simulink model "mdl_VD_st2dof_R2025b_SLX"  (R2025b)
settings: Solver=ode3  StartTime=startTime  StopTime=endTime  FixedStep=deltaT  MaxStep=deltaT  RelTol=1e-3  EnableMultiTasking=on
values from neighbouring files (symbols this model uses):
  initialStates = [0 0 0 0 0]    [script_test_fcn_VD_st2dofSimulink.m]
  parameters = struct    [fcn_VD_st2dofSimulink.m]
  U = 20    [script_test_fcn_VD_st2dofSimulink.m]
settings Model: Creator=snb10  LastModifiedBy=snb10
settings SolverCC: AlgebraicLoopSolver=TrustRegion
settings DataIOCC: LimitDataPoints=on  SaveFormat=Array  SignalLoggingSaveFormat=ModelDataLogs  ReturnWorkspaceOutputs=off  SignalLoggingName=sigsOut
settings OptimizationCC: InitFltsAndDblsToZero=on  LifeSpan=inf
settings DebuggingCC: SaveWithParameterizedLinksMsg=none  UnderspecifiedInitializationDetection=Classic  MergeDetectMultiDrivingBlocksExec=none  SignalResolutionControl=TryResolveAllWithWarning  MultiTaskDSMMsg=warning  MultiTaskCondExecSysMsg=none  FcnCallInpInsideContextMsg=warning  UnconnectedInputMsg=warning  UnconnectedOutputMsg=warning  UnconnectedLineMsg=warning  StateNameClashWarn=warning  SFUnexpectedBacktrackingDiag=warning  SFNoUnconditionalDefaultTransitionDiag=warning  SFExecutionAtInitializationDiag=none  ArithmeticOperatorsInVariantConditions=warning
settings HardwareCC: ProdBitPerPointer=32.0  ProdBitPerSizeT=32.0  ProdBitPerPtrDiffT=32.0  ProdLargestAtomicFloat=None  ProdIntDivRoundTo=Undefined  ProdEndianess=Unspecified  ProdWordSize=32.0  ProdHWDeviceType=32-bit Generic  TargetUnknown=on
settings ModelReferenceCC: EnableRefExpFcnMdlSchedulingChecks=on  PropagateSignalLabelsOutOfModel=off
settings SFSimCC: SimUseLocalCustomCode=off  CustomCodeUndefinedFunction=UseInterfaceOnly
settings RTWCC: RTWUseLocalCustomCode=off  GPUComputeCapability=3.5  DLArmComputeVersion=19.05
settings CodeAppCC: StateflowObjectComments=on
settings GRTTargetCC: TargetFcnLib=ansi_tfl_tmw.mat  TargetLangStandard=C89/C90 (ANSI)  CombineOutputUpdateFcns=off  GRTInterface=on
settings ConfigComp: CovMetricSettings=dw  CovSaveCumulativeToWorkspaceVar=on  CovSaveSingleToWorkspaceVar=on  CovExternalEMLEnable=off

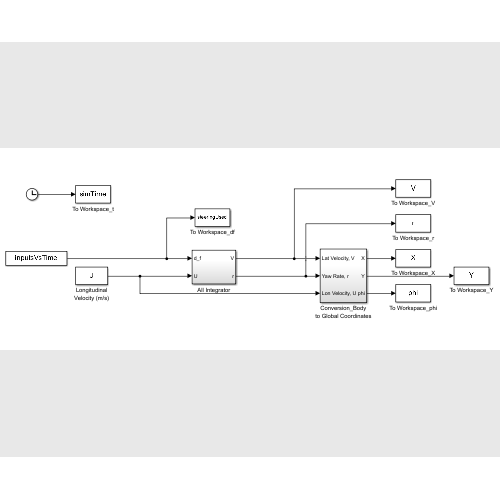
[thumbnail: Simulink's stored preview of the top-level diagram]
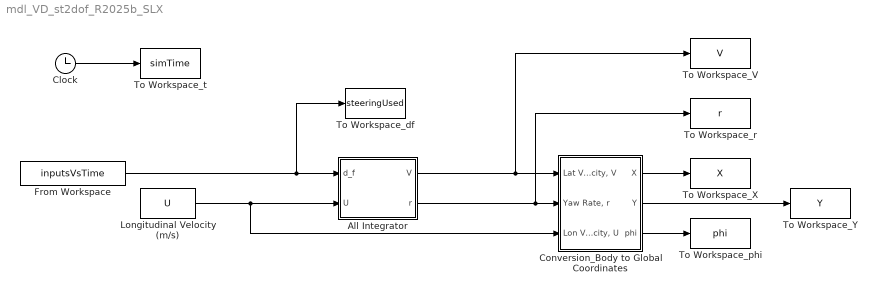
== system mdl_VD_st2dof_R2025b_SLX ==
  All Integrator : Subsystem
  Clock : Clock
  Conversion_Body to Global Coordinates : Subsystem
  From Workspace : FromWorkspace  VariableName=inputsVsTime  OutDataTypeStr=double  SampleTime=.01  OutputAfterFinalValue=Holding final value
  Longitudinal Velocity (m/s) : Constant  Value=U
  To Workspace_V : ToWorkspace  VariableName=V  SampleTime=-1
  To Workspace_X : ToWorkspace  VariableName=X  SampleTime=-1
  To Workspace_Y : ToWorkspace  VariableName=Y  SampleTime=-1
  To Workspace_df : ToWorkspace  VariableName=steeringUsed  SampleTime=-1
  To Workspace_phi : ToWorkspace  VariableName=phi  SampleTime=-1
  To Workspace_r : ToWorkspace  VariableName=r  SampleTime=-1
  To Workspace_t : ToWorkspace  VariableName=simTime  SampleTime=-1
  wires:
  Clock/1 -> To Workspace_t/1
  All Integrator/1(V) -> Conversion_Body to Global Coordinates/1("Lat Velocity, V"), To Workspace_V/1
  Conversion_Body to Global Coordinates/1(X) -> To Workspace_X/1
  Conversion_Body to Global Coordinates/2(Y) -> To Workspace_Y/1
  All Integrator/2(r) -> Conversion_Body to Global Coordinates/2("Yaw Rate, r"), To Workspace_r/1
  Conversion_Body to Global Coordinates/3(phi) -> To Workspace_phi/1
  Longitudinal Velocity (m/s)/1 -> Conversion_Body to Global Coordinates/3("Lon Velocity, U"), All Integrator/2(U)
  From Workspace/1 -> To Workspace_df/1, All Integrator/1(d_f)

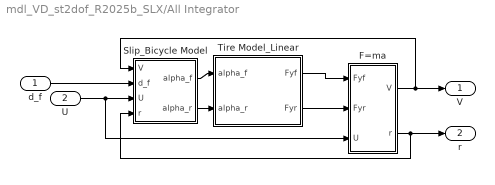
== system mdl_VD_st2dof_R2025b_SLX/All Integrator ==
  d_f : Inport
  U : Inport  Port=2
  F=ma : Subsystem
  Slip_Bicycle Model : Subsystem
  Tire Model_Linear : Subsystem
  V : Outport
  r : Outport  Port=2
  wires:
  Slip_Bicycle Model/1(alpha_f) -> Tire Model_Linear/1(alpha_f)
  Slip_Bicycle Model/2(alpha_r) -> Tire Model_Linear/2(alpha_r)
  Tire Model_Linear/1(Fyf) -> F=ma/1(Fyf)
  Tire Model_Linear/2(Fyr) -> F=ma/2(Fyr)
  U/1 -> Slip_Bicycle Model/3(U), F=ma/3(" U")
  d_f/1 -> Slip_Bicycle Model/2(d_f)
  F=ma/1(V) -> V/1, Slip_Bicycle Model/1(V)
  F=ma/2(r) -> r/1, Slip_Bicycle Model/4(r)

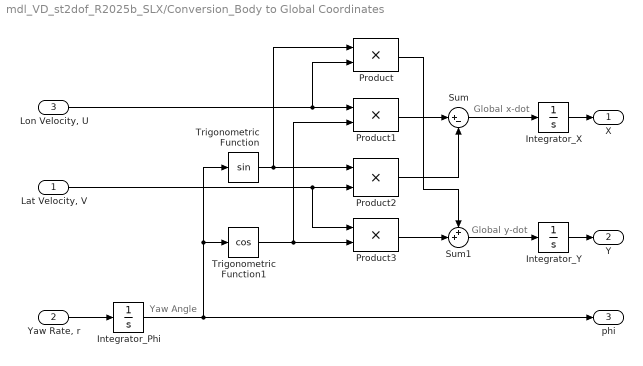
== system mdl_VD_st2dof_R2025b_SLX/Conversion_Body to Global Coordinates ==
  note: Global y-dot
  note: Global x-dot
  note: Yaw Angle
  "Lat Velocity, V" : Inport
  "Yaw Rate, r" : Inport  Port=2
  "Lon Velocity, U" : Inport  Port=3
  Integrator_Phi : Integrator  InitialCondition=initialStates(5)
  Integrator_X : Integrator  InitialCondition=initialStates(3)
  Integrator_Y : Integrator  InitialCondition=initialStates(4)
  Product{,1..3} (4 alike) : Product  SaturateOnIntegerOverflow=on  OutDataTypeStr=Inherit: Same as first input
  Sum : Sum  Inputs=|+-  SaturateOnIntegerOverflow=on
  Sum1 : Sum  Inputs=++|  SaturateOnIntegerOverflow=on
  Trigonometric Function : Trigonometry
  Trigonometric Function1 : Trigonometry  Operator=cos
  X : Outport
  Y : Outport  Port=2
  phi : Outport  Port=3
  wires:
  Integrator_Y/1 -> Y/1
  Integrator_X/1 -> X/1
  "Yaw Rate, r"/1 -> Integrator_Phi/1
  Sum1/1 -> Integrator_Y/1
  Product3/1 -> Sum1/2
  Product/1 -> Sum1/1
  Sum/1 -> Integrator_X/1
  Trigonometric Function/1 -> Product/1, Product2/1
  Product2/1 -> Sum/2
  Product1/1 -> Sum/1
  Trigonometric Function1/1 -> Product1/2, Product3/2
  "Lat Velocity, V"/1 -> Product3/1, Product2/2
  "Lon Velocity, U"/1 -> Product/2, Product1/1
  Integrator_Phi/1 -> phi/1, Trigonometric Function/1, Trigonometric Function1/1

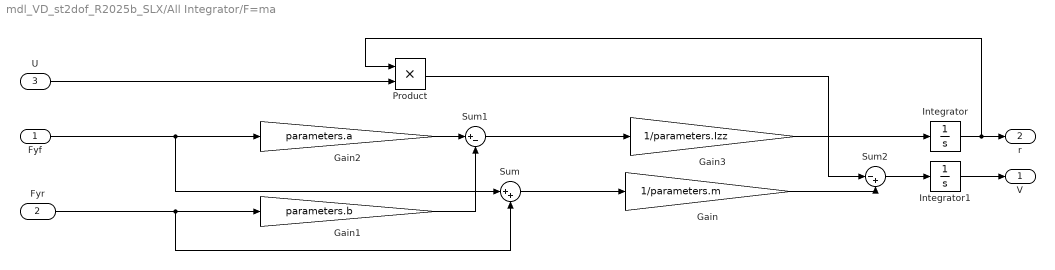
== system mdl_VD_st2dof_R2025b_SLX/All Integrator/F=ma ==
  Fyf : Inport
  Fyr : Inport  Port=2
  " U" : Inport  Port=3
  Gain : Gain  Gain=1/parameters.m
  Gain1 : Gain  Gain=parameters.b
  Gain2 : Gain  Gain=parameters.a
  Gain3 : Gain  Gain=1/parameters.Izz
  Integrator : Integrator  InitialCondition=initialStates(1)
  Integrator1 : Integrator  InitialCondition=initialStates(2)
  Product : Product  RndMeth=Zero
  Sum : Sum  Inputs=|++
  Sum1 : Sum  Inputs=|+-
  Sum2 : Sum  Inputs=|-+
  V : Outport
  r : Outport  Port=2
  wires:
  Fyf/1 -> Sum/1, Gain2/1
  Fyr/1 -> Sum/2, Gain1/1
  Gain2/1 -> Sum1/1
  Gain1/1 -> Sum1/2
  Sum1/1 -> Gain3/1
  Gain3/1 -> Integrator/1
  Sum/1 -> Gain/1
  Product/1 -> Sum2/1
  Gain/1 -> Sum2/2
  Sum2/1 -> Integrator1/1
  Integrator/1 -> r/1, Product/1
  Integrator1/1 -> V/1
  " U"/1 -> Product/2

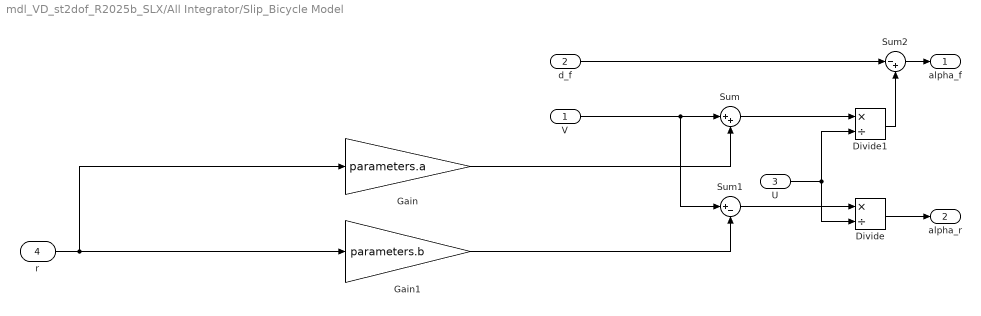
== system mdl_VD_st2dof_R2025b_SLX/All Integrator/Slip_Bicycle Model ==
  V : Inport
  d_f : Inport  Port=2
  U : Inport  Port=3
  r : Inport  Port=4
  Divide : Product  Inputs=*/
  Divide1 : Product  Inputs=*/
  Gain : Gain  Gain=parameters.a
  Gain1 : Gain  Gain=parameters.b
  Sum : Sum  Inputs=|++
  Sum1 : Sum  Inputs=|+-
  Sum2 : Sum  Inputs=|-+
  alpha_f : Outport
  alpha_r : Outport  Port=2
  wires:
  V/1 -> Sum/1, Sum1/1
  Gain/1 -> Sum/2
  r/1 -> Gain/1, Gain1/1
  Gain1/1 -> Sum1/2
  Sum/1 -> Divide1/1
  U/1 -> Divide1/2, Divide/2
  Sum1/1 -> Divide/1
  Divide1/1 -> Sum2/2
  d_f/1 -> Sum2/1
  Sum2/1 -> alpha_f/1
  Divide/1 -> alpha_r/1

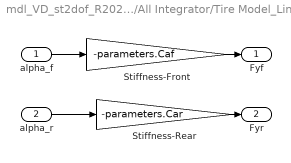
== system mdl_VD_st2dof_R2025b_SLX/All Integrator/Tire Model_Linear ==
  alpha_f : Inport
  alpha_r : Inport  Port=2
  Stiffness-Front : Gain  Gain=-parameters.Caf
  Stiffness-Rear : Gain  Gain=-parameters.Car
  Fyf : Outport
  Fyr : Outport  Port=2
  wires:
  alpha_f/1 -> Stiffness-Front/1
  Stiffness-Front/1 -> Fyf/1
  alpha_r/1 -> Stiffness-Rear/1
  Stiffness-Rear/1 -> Fyr/1
